simulink library "ConverterLibrary"  (R2026a)
settings: Solver=VariableStepAuto
undefined symbols (not defined in the file or in its folder): DiscIntNeverNeededParam, dspblkCoreblockFVToolHelper, gcbh, gridInverter
libraries: fl_lib x240, nesl_utility x221, ee_lib x208, slpidlib x28, eeGeneralControl x12, simulink x9, eeTransforms x4, simulink_extras x1, eePowerMeasurement x1
(part 6 of 30)

== system ConverterLibrary/Controller/Inverter-Based Resources/Grid-Forming Converter Controller/Measurement ==
  Vgabcc : Inport
  Igabc : Inport  Port=2
  Angle : Inport  Port=3
  Frequency Measurement : Subsystem
  Gain1 : Gain  Gain=1/power
  Gain2 : Gain  Gain=1/power
  Gain3 : Gain  Gain=gridLineVoltage*sqrt(2/3)
  Gain4 : Gain  Gain=gridLineVoltage*sqrt(2/3)
  Gain5 : Gain  Gain=power/(sqrt(3)*gridLineVoltage)*sqrt(2)
  PU2Hz : Gain  Gain=gridInverter.frequency
  Power Measurement (Three-Phase)1 : eePowerMeasurement/Power Measurement (Three-Phase)  LabelModeActiveChoice=Discrete  F=powerFreq  K=[1]  Seq=Positive  Ts=measSampleTime
  abc2dq : Subsystem
  Out Bus Element : Outport  PortName=measure  Element=P
  Out Bus Element1 : Outport  PortName=measure  Element=Q
  Out Bus Element2 : Outport  PortName=measure  Element=Vgd
  Out Bus Element3 : Outport  PortName=measure  Element=Vgq
  Out Bus Element4 : Outport  PortName=measure  Element=Igd
  Out Bus Element5 : Outport  PortName=measure  Element=Igq
  Out Bus Element6 : Outport  PortName=measure  Element=fgrid
  PmeasPU : Outport  Port=2
  QmeasPU : Outport  Port=3
  FmeasHz : Outport  Port=4
  wires:
  Gain3/1 -> Frequency Measurement/1(Vabc)  "Vgd"
  Gain1/1 -> Out Bus Element1/1, QmeasPU/1  "Qmeas"
  Gain2/1 -> PmeasPU/1, Out Bus Element/1  "Pmeas"
  Gain5/1 -> Power Measurement (Three-Phase)1/2  "Igd"
  Gain4/1 -> Power Measurement (Three-Phase)1/1  "Vgd"
  Power Measurement (Three-Phase)1/2 -> Gain1/1  "Qmeas"
  Power Measurement (Three-Phase)1/1 -> Gain2/1  "Pmeas"
  PU2Hz/1 -> FmeasHz/1
  Frequency Measurement/1(freq) -> Out Bus Element6/1, PU2Hz/1
  abc2dq/4(Igq) -> Out Bus Element5/1  "Igq"
  abc2dq/3(Igd) -> Out Bus Element4/1  "Igd"
  abc2dq/1(Vgd) -> Out Bus Element2/1  "Vgd"
  abc2dq/2(Vgq) -> Out Bus Element3/1  "Vgq"
  Igabc/1 -> abc2dq/1(Igabc), Gain5/1  "Iabc"
  Angle/1 -> abc2dq/2(Angle)
  Vgabcc/1 -> Gain4/1, Gain3/1, abc2dq/3(Vgabc)  "Vabc"

== system ConverterLibrary/Controller/Inverter-Based Resources/Grid-Forming Converter Controller/Power Control ==
  note: Active Power Control
  note: Reactive Power Control
  In Bus Element2 : Inport  PortName=measure  Element=P
  In Bus Element3 : Inport  PortName=measure  Element=Q
  In Bus Element1 : Inport  PortName=measure  Element=fgrid
  Pref : Inport  Port=2
  Qref : Inport  Port=3
  ActivePowerControl : Subsystem  Variant=on  VariantControlMode=label  VariantControl=Choice  LabelModeActiveChoice=vsm
  ReactiveControl : Subsystem
  Out Bus Element : Outport  PortName=reactiveControl  Element=Vmd
  Out Bus Element1 : Outport  PortName=reactiveControl  Element=Vmq
  Out Bus Element6 : Outport  Port=2  PortName=activeControl  Element=angle
  Out Bus Element4 : Outport  Port=2  PortName=activeControl  Element=w
  angle : Outport  Port=3
  wires:
  In Bus Element1/1 -> ActivePowerControl/3(fgrid)
  In Bus Element2/1 -> ActivePowerControl/2(Pmeas)
  Qref/1 -> ReactiveControl/1(Qref)  "Q"
  Pref/1 -> ActivePowerControl/1(Pref)  "Q"
  ReactiveControl/2(Vmq) -> Out Bus Element1/1
  ReactiveControl/1(Vmd) -> Out Bus Element/1
  ActivePowerControl/1(Theta) -> Out Bus Element6/1, angle/1
  In Bus Element3/1 -> ReactiveControl/2(Qmeas)
  ActivePowerControl/2(w) -> Out Bus Element4/1

== system ConverterLibrary/Controller/Inverter-Based Resources/Grid-Forming Converter Controller/VoltageCurrentControl ==
  In Bus Element : Inport  PortName=currentLimiting  Element=Vmd
  In Bus Element1 : Inport  PortName=currentLimiting  Element=Vmq
  In Bus Element6 : Inport  PortName=currentLimiting  Element=Idmax
  In Bus Element7 : Inport  PortName=currentLimiting  Element=Iqmax
  Bus Element In6 : Inport  Port=2  PortName=activeControl  Element=w
  Bus Element In1 : Inport  Port=2  PortName=activeControl  Element=angle
  In Bus Element2 : Inport  Port=3  PortName=measure  Element=Vgd
  In Bus Element3 : Inport  Port=3  PortName=measure  Element=Vgq
  In Bus Element4 : Inport  Port=3  PortName=measure  Element=Igd
  In Bus Element5 : Inport  Port=3  PortName=measure  Element=Igq
  Controller : Subsystem
  Modulation Signal : Subsystem
  mabc : Outport
  wires:
  Bus Element In1/1 -> Modulation Signal/3(Angle)
  In Bus Element1/1 -> Controller/3(Vgqref)
  In Bus Element/1 -> Controller/2(Vgdref)
  Bus Element In6/1 -> Controller/1(Angfreq)
  In Bus Element3/1 -> Controller/5(Vsq)
  In Bus Element2/1 -> Controller/4(Vsd)
  In Bus Element7/1 -> Controller/9(Iqmax)
  In Bus Element6/1 -> Controller/8(Idmax)
  In Bus Element5/1 -> Controller/7(Iq)
  In Bus Element4/1 -> Controller/6(Id)
  Controller/1(Vd) -> Modulation Signal/1(Vd)
  Modulation Signal/1(mabc) -> mabc/1
  Controller/2(Vq) -> Modulation Signal/2(Vq)

== system ConverterLibrary/Controller/Non-Isolated DC-DC Converters/Non-Isolated DC-DC Controller/Duty Feedforward ==
  voltageReferencePu : Inport
  inputVoltagePuOut : Inport  Port=2
  Duty Max : Constant  Value=dutyMax
  Duty Min : Constant  Value=dutyMin
  Feedforward Law : Subsystem  Variant=on  VariantControlMode=label  LabelModeActiveChoice=Boost
  Feedforward Limit : Saturate  UpperLimit=dutyMax  LowerLimit=dutyMin
  Input Clamp : Saturate  UpperLimit=inf  LowerLimit=inputVoltagePuMin
  Reference Clamp : Saturate  UpperLimit=inf  LowerLimit=voltageReferencePuMin
  Sum : Sum  Inputs=|+-
  Sum1 : Sum  Inputs=|-+
  trimUpperLimit : Outport
  trimLowerLimit : Outport  Port=2
  dutyFeedforward : Outport  Port=3
  wires:
  Feedforward Limit/1 -> dutyFeedforward/1, Sum1/1, Sum/2
  Feedforward Law/1(dutyFeedforward) -> Feedforward Limit/1
  Input Clamp/1 -> Feedforward Law/2(inputVoltagePuOut)
  Reference Clamp/1 -> Feedforward Law/1(voltageReferencePu)
  inputVoltagePuOut/1 -> Input Clamp/1
  voltageReferencePu/1 -> Reference Clamp/1
  Duty Max/1 -> Sum/1
  Sum/1 -> trimUpperLimit/1
  Sum1/1 -> trimLowerLimit/1
  Duty Min/1 -> Sum1/2

== system ConverterLibrary/Controller/Non-Isolated DC-DC Converters/Non-Isolated DC-DC Controller/Loop Structure ==
  voltageControllerOutput : Inport
  inductorCurrentPu : Inport  Port=2
  trimUpperLimit : Inport  Port=3
  trimLowerLimit : Inport  Port=4
  DoubleLoop : Subsystem  VariantControl=DoubleLoop
  SingleLoop : Subsystem  VariantControl=SingleLoop
  dutyTrim : Outport

== system ConverterLibrary/Controller/Non-Isolated DC-DC Converters/Non-Isolated DC-DC Controller/Output Mode ==
  duty : Inport
  DutyCycle : Subsystem  VariantControl=DutyCycle
  PWMSignal : Subsystem  VariantControl=PWMSignal
  G : Outport

== system ConverterLibrary/Controller/Non-Isolated DC-DC Converters/Non-Isolated DC-DC Controller/Per-Unit Scaling ==
  Vref : Inport
  Vmeas : Inport  Port=2
  Imeas : Inport  Port=3
  Vin : Inport  Port=4
  Imeas ADC Sample : UnitDelay  SampleTime=TsCurrent
  Imeas Inductor Base : Gain  Gain=1/IbaseL
  Vin ADC Sample : UnitDelay  InitialCondition=VbaseIn  SampleTime=TsVoltage
  Vin Output Base : Gain  Gain=1/VbaseOut
  Vmeas ADC Sample : UnitDelay  SampleTime=TsVoltage
  Vmeas Output Base : Gain  Gain=1/VbaseOut
  Vref Output Base : Gain  Gain=1/VbaseOut
  outputVoltagePu : Outport
  voltageReferencePu : Outport  Port=2
  inductorCurrentPu : Outport  Port=3
  inputVoltagePuOut : Outport  Port=4
  wires:
  Vin Output Base/1 -> inputVoltagePuOut/1
  Vin ADC Sample/1 -> Vin Output Base/1
  Vin/1 -> Vin ADC Sample/1
  Imeas Inductor Base/1 -> inductorCurrentPu/1
  Imeas ADC Sample/1 -> Imeas Inductor Base/1
  Imeas/1 -> Imeas ADC Sample/1
  Vmeas Output Base/1 -> outputVoltagePu/1
  Vmeas ADC Sample/1 -> Vmeas Output Base/1
  Vmeas/1 -> Vmeas ADC Sample/1
  Vref Output Base/1 -> voltageReferencePu/1
  Vref/1 -> Vref Output Base/1

== system ConverterLibrary/Controller/Non-Isolated DC-DC Converters/Non-Isolated DC-DC Controller/Voltage Controller ==
  error : Inport
  PIContinuous : Subsystem  VariantControl=PIContinuous
  PIDiscrete : Subsystem  VariantControl=PIDiscrete
  vc : Outport

== system ConverterLibrary/Controller/PWM Generators/CLLC PWM Generator/Primary Gate Signal ==
  fpu : Inport
  Bridge Gate Map : Selector  InputPortWidth=2  IndexOptions=Index vector (dialog)  Indices=[1 2 2 1]  OutputSizes=1
  Dead Time : Constant  Value=Tdead
  Gate Level Offset : Bias  Bias=gateVoltageOff
  Gate Level Swing : Gain  Gain=gateVoltageOn - gateVoltageOff
  Hertz To Period : Math  Operator=reciprocal
  Leg Gate Logic : Subsystem
  Normalized To Hertz : Gain  Gain=Fbase
  Primary Gates To Logic : DataTypeConversion  OutDataTypeStr=boolean
  Pulse Time : Gain  Gain=pulseWidth
  Pulse Time Plus Dead Time : Bias  Bias=Tdead
  Ramp Mode : Subsystem  Variant=on  VariantControlMode=label  LabelModeActiveChoice=VariableStep
  Turn Off Times : Mux  Inputs=2
  Turn On Times : Mux  Inputs=2
  G : Outport
  gates : Outport  Port=2
  wires:
  Gate Level Swing/1 -> Gate Level Offset/1
  fpu/1 -> Normalized To Hertz/1
  Normalized To Hertz/1 -> Hertz To Period/1
  Hertz To Period/1 -> Pulse Time/1, Turn Off Times/2, Ramp Mode/1(Tsw)
  Pulse Time/1 -> Pulse Time Plus Dead Time/1, Turn Off Times/1
  Dead Time/1 -> Turn On Times/1
  Pulse Time Plus Dead Time/1 -> Turn On Times/2
  Turn On Times/1 -> Leg Gate Logic/1(Ton)
  Turn Off Times/1 -> Leg Gate Logic/2(Toff)
  Ramp Mode/1(S) -> Leg Gate Logic/3(S)
  Leg Gate Logic/1(gates) -> Bridge Gate Map/1
  Bridge Gate Map/1 -> Gate Level Swing/1, Primary Gates To Logic/1
  Gate Level Offset/1 -> G/1
  Primary Gates To Logic/1 -> gates/1

== system ConverterLibrary/Controller/PWM Generators/CLLC PWM Generator/Synchronous Rectifier ==
  primaryGates : Inport
  fpu : Inport  Port=2
  Isec : Inport  Port=3
  Conduction Detect : Subsystem
  Rectifier Gate Level Offset : Bias  Bias=srGateVoltageOff
  Rectifier Gate Level Swing : Gain  Gain=srGateVoltageOn - srGateVoltageOff
  Rectifier Gates To Double : DataTypeConversion  OutDataTypeStr=double
  Region Select : Subsystem
  Turn On Delay : Subsystem
  Gs : Outport
  wires:
  Rectifier Gate Level Swing/1 -> Rectifier Gate Level Offset/1
  primaryGates/1 -> Region Select/1(primaryGates)
  fpu/1 -> Region Select/2(fpu)
  Isec/1 -> Conduction Detect/1(Isec)
  Conduction Detect/1(permit) -> Region Select/3(permit)
  Region Select/1(Gs) -> Turn On Delay/1(condition)
  Turn On Delay/1(Gs) -> Rectifier Gates To Double/1
  Rectifier Gates To Double/1 -> Rectifier Gate Level Swing/1
  Rectifier Gate Level Offset/1 -> Gs/1

== system ConverterLibrary/Controller/PWM Generators/Complementary PWM Generator/Ramp Mode ==
  rate : Inport
  FixedStep : Subsystem  VariantControl=FixedStep
  VariableStep : Subsystem  VariantControl=VariableStep
  S : Outport

== system ConverterLibrary/Controller/PWM Generators/DAB PWM Generator/Primary Leg Gate Logic ==
  Ton : Inport
  Toff : Inport  Port=2
  S : Inport  Port=3
  After Turn Off : RelationalOperator
  After Turn On : RelationalOperator
  Pulse Window : Logic  Operator=XOR
  To Double : DataTypeConversion  OutDataTypeStr=double
  gates : Outport
  wires:
  Ton/1 -> After Turn On/2
  Toff/1 -> After Turn Off/2
  S/1 -> After Turn Off/1, After Turn On/1
  After Turn On/1 -> Pulse Window/1
  After Turn Off/1 -> Pulse Window/2
  Pulse Window/1 -> To Double/1
  To Double/1 -> gates/1

== system ConverterLibrary/Controller/PWM Generators/DAB PWM Generator/Ramp Mode ==
  Tsw : Inport
  FixedStep : Subsystem  VariantControl=FixedStep
  VariableStep : Subsystem  VariantControl=VariableStep
  S : Outport

== system ConverterLibrary/Controller/PWM Generators/DAB PWM Generator/Secondary Leg Gate Logic ==
  Ton : Inport
  Toff : Inport  Port=2
  S : Inport  Port=3
  After Turn Off : RelationalOperator
  After Turn On : RelationalOperator
  Pulse Window : Logic  Operator=XOR
  To Double : DataTypeConversion  OutDataTypeStr=double
  gates : Outport
  wires:
  Ton/1 -> After Turn On/2
  Toff/1 -> After Turn Off/2
  S/1 -> After Turn Off/1, After Turn On/1
  After Turn On/1 -> Pulse Window/1
  After Turn Off/1 -> Pulse Window/2
  Pulse Window/1 -> To Double/1
  To Double/1 -> gates/1

== system ConverterLibrary/Controller/PWM Generators/Full Bridge PWM Generator/Leg Gate Logic ==
  Ton : Inport
  Toff : Inport  Port=2
  S : Inport  Port=3
  After Turn Off : RelationalOperator
  After Turn On : RelationalOperator
  Pulse Window : Logic  Operator=XOR
  To Double : DataTypeConversion  OutDataTypeStr=double
  gates : Outport
  wires:
  Ton/1 -> After Turn On/2
  Toff/1 -> After Turn Off/2
  S/1 -> After Turn Off/1, After Turn On/1
  After Turn On/1 -> Pulse Window/1
  After Turn Off/1 -> Pulse Window/2
  Pulse Window/1 -> To Double/1
  To Double/1 -> gates/1

== system ConverterLibrary/Controller/PWM Generators/Full Bridge PWM Generator/Ramp Mode ==
  Tsw : Inport
  FixedStep : Subsystem  VariantControl=FixedStep
  VariableStep : Subsystem  VariantControl=VariableStep
  S : Outport

== system ConverterLibrary/Controller/PWM Generators/Half Bridge PWM Generator/Leg Gate Logic ==
  Ton : Inport
  Toff : Inport  Port=2
  S : Inport  Port=3
  After Turn Off : RelationalOperator
  After Turn On : RelationalOperator
  Pulse Window : Logic  Operator=XOR
  To Double : DataTypeConversion  OutDataTypeStr=double
  gates : Outport
  wires:
  Ton/1 -> After Turn On/2
  Toff/1 -> After Turn Off/2
  S/1 -> After Turn Off/1, After Turn On/1
  After Turn On/1 -> Pulse Window/1
  After Turn Off/1 -> Pulse Window/2
  Pulse Window/1 -> To Double/1
  To Double/1 -> gates/1

== system ConverterLibrary/Controller/PWM Generators/Half Bridge PWM Generator/Ramp Mode ==
  Tsw : Inport
  FixedStep : Subsystem  VariantControl=FixedStep
  VariableStep : Subsystem  VariantControl=VariableStep
  S : Outport

== system ConverterLibrary/Controller/PWM Generators/LLC PWM Generator/Leg Gate Logic ==
  Ton : Inport
  Toff : Inport  Port=2
  S : Inport  Port=3
  After Turn Off : RelationalOperator
  After Turn On : RelationalOperator
  Pulse Window : Logic  Operator=XOR
  To Double : DataTypeConversion  OutDataTypeStr=double
  gates : Outport
  wires:
  Ton/1 -> After Turn On/2
  Toff/1 -> After Turn Off/2
  S/1 -> After Turn Off/1, After Turn On/1
  After Turn On/1 -> Pulse Window/1
  After Turn Off/1 -> Pulse Window/2
  Pulse Window/1 -> To Double/1
  To Double/1 -> gates/1

== system ConverterLibrary/Controller/PWM Generators/LLC PWM Generator/Ramp Mode ==
  Tsw : Inport
  FixedStep : Subsystem  VariantControl=FixedStep
  VariableStep : Subsystem  VariantControl=VariableStep
  S : Outport

== system ConverterLibrary/Controller/Power Factor Correction Converters/Boost PFC Controller/Current Controller ==
  error : Inport
  up : Inport  Port=2
  lo : Inport  Port=3
  PIContinuous : Subsystem  VariantControl=PIContinuous
  PIDiscrete : Subsystem  VariantControl=PIDiscrete
  vc : Outport

== system ConverterLibrary/Controller/Power Factor Correction Converters/Boost PFC Controller/Duty Feedforward ==
  busVoltagePuDC : Inport
  absLineVoltagePuDC : Inport  Port=2
  Bus Clamp : Saturate  UpperLimit=inf  LowerLimit=VacPeakPuDC
  Duty Max : Constant  Value=dutyMax
  Duty Min : Constant  Value=dutyMin
  Feedforward One : Constant
  Feedforward Ratio : Product  Inputs=*/
  One Minus Ratio : Sum  Inputs=|+-
  Trim Lower Limit : Sum  Inputs=|+-
  Trim Upper Limit : Sum  Inputs=|+-
  trimUpperLimit : Outport
  trimLowerLimit : Outport  Port=2
  dutyFeedforward : Outport  Port=3
  wires:
  Trim Lower Limit/1 -> trimLowerLimit/1
  Trim Upper Limit/1 -> trimUpperLimit/1
  Duty Min/1 -> Trim Lower Limit/1
  Duty Max/1 -> Trim Upper Limit/1
  One Minus Ratio/1 -> Trim Lower Limit/2, Trim Upper Limit/2, dutyFeedforward/1
  Feedforward Ratio/1 -> One Minus Ratio/2
  Feedforward One/1 -> One Minus Ratio/1
  Bus Clamp/1 -> Feedforward Ratio/2
  absLineVoltagePuDC/1 -> Feedforward Ratio/1
  busVoltagePuDC/1 -> Bus Clamp/1

== system ConverterLibrary/Controller/Power Factor Correction Converters/Boost PFC Controller/Output Mode ==
  duty : Inport
  DutyCycle : Subsystem  VariantControl=DutyCycle
  PWMSignal : Subsystem  VariantControl=PWMSignal
  G : Outport

== system ConverterLibrary/Controller/Power Factor Correction Converters/Boost PFC Controller/Per-Unit Scaling ==
  Vac : Inport
  Vref : Inport  Port=2
  Vmeas : Inport  Port=3
  IL : Inport  Port=4
  Abs Line Current : Abs  SaturateOnIntegerOverflow=off
  Abs Vac : Abs  SaturateOnIntegerOverflow=off
  Abs Vac AC Base : Gain  Gain=1/VbaseAC
  Abs Vac DC Base : Gain  Gain=1/VbaseDC
  IL AC Base : Gain  Gain=1/IbaseAC
  IL ADC Sample : UnitDelay  SampleTime=TsCurrent
  Vac ADC Sample : UnitDelay  SampleTime=TsCurrent
  Vmeas ADC Sample : UnitDelay  SampleTime=TsVoltage
  Vmeas DC Base : Gain  Gain=1/VbaseDC
  Vref DC Base : Gain  Gain=1/VbaseDC
  absLineVoltagePuAC : Outport
  voltageReferencePuDC : Outport  Port=2
  busVoltagePuDC : Outport  Port=3
  absLineCurrentPuAC : Outport  Port=4
  absLineVoltagePuDC : Outport  Port=5
  wires:
  Abs Line Current/1 -> absLineCurrentPuAC/1
  IL AC Base/1 -> Abs Line Current/1
  IL ADC Sample/1 -> IL AC Base/1
  IL/1 -> IL ADC Sample/1
  Vmeas DC Base/1 -> busVoltagePuDC/1
  Vmeas ADC Sample/1 -> Vmeas DC Base/1
  Vmeas/1 -> Vmeas ADC Sample/1
  Vref DC Base/1 -> voltageReferencePuDC/1
  Vref/1 -> Vref DC Base/1
  Abs Vac DC Base/1 -> absLineVoltagePuDC/1
  Abs Vac AC Base/1 -> absLineVoltagePuAC/1
  Abs Vac/1 -> Abs Vac AC Base/1, Abs Vac DC Base/1
  Vac ADC Sample/1 -> Abs Vac/1
  Vac/1 -> Vac ADC Sample/1

== system ConverterLibrary/Controller/Power Factor Correction Converters/Boost PFC Controller/Voltage Controller ==
  error : Inport
  PIContinuous : Subsystem  VariantControl=PIContinuous
  PIDiscrete : Subsystem  VariantControl=PIDiscrete
  vc : Outport

== system ConverterLibrary/Controller/Power Factor Correction Converters/Interleaved Boost PFC Controller/Current Balance ==
  leg1CurrentPuAC : Inport
  leg2CurrentPuAC : Inport  Port=2
  Balance Controller : Subsystem  Variant=on  VariantControlMode=label  LabelModeActiveChoice=PIContinuous
  Half Difference : Gain  Gain=0.5
  Leg Current Difference : Sum  Inputs=|+-
  dutyTrim : Outport
  wires:
  Balance Controller/1(vc) -> dutyTrim/1
  Half Difference/1 -> Balance Controller/1(error)
  Leg Current Difference/1 -> Half Difference/1
  leg2CurrentPuAC/1 -> Leg Current Difference/2
  leg1CurrentPuAC/1 -> Leg Current Difference/1

== system ConverterLibrary/Controller/Power Factor Correction Converters/Interleaved Boost PFC Controller/Current Controller ==
  error : Inport
  up : Inport  Port=2
  lo : Inport  Port=3
  PIContinuous : Subsystem  VariantControl=PIContinuous
  PIDiscrete : Subsystem  VariantControl=PIDiscrete
  vc : Outport

== system ConverterLibrary/Controller/Power Factor Correction Converters/Interleaved Boost PFC Controller/Duty Feedforward ==
  busVoltagePuDC : Inport
  absLineVoltagePuDC : Inport  Port=2
  Bus Clamp : Saturate  UpperLimit=inf  LowerLimit=VacPeakPuDC
  Duty Max : Constant  Value=dutyMax
  Duty Min : Constant  Value=dutyMin
  Feedforward One : Constant
  Feedforward Ratio : Product  Inputs=*/
  One Minus Ratio : Sum  Inputs=|+-
  Trim Lower Limit : Sum  Inputs=|+-
  Trim Upper Limit : Sum  Inputs=|+-
  trimUpperLimit : Outport
  trimLowerLimit : Outport  Port=2
  dutyFeedforward : Outport  Port=3
  wires:
  Trim Lower Limit/1 -> trimLowerLimit/1
  Trim Upper Limit/1 -> trimUpperLimit/1
  Duty Min/1 -> Trim Lower Limit/1
  Duty Max/1 -> Trim Upper Limit/1
  One Minus Ratio/1 -> dutyFeedforward/1, Trim Upper Limit/2, Trim Lower Limit/2
  Feedforward Ratio/1 -> One Minus Ratio/2
  Feedforward One/1 -> One Minus Ratio/1
  Bus Clamp/1 -> Feedforward Ratio/2
  absLineVoltagePuDC/1 -> Feedforward Ratio/1
  busVoltagePuDC/1 -> Bus Clamp/1

== system ConverterLibrary/Controller/Power Factor Correction Converters/Interleaved Boost PFC Controller/Duty Split ==
  dutyCommon : Inport
  dutyTrim : Inport  Port=2
  Leg 1 Duty : Sum  Inputs=|+-
  Leg 1 Duty Limit : Saturate  UpperLimit=dutyMax  LowerLimit=dutyMin
  Leg 2 Duty : Sum  Inputs=|++
  Leg 2 Duty Limit : Saturate  UpperLimit=dutyMax  LowerLimit=dutyMin
  Leg Duties : Mux  Inputs=2
  duty : Outport
  wires:
  Leg Duties/1 -> duty/1
  Leg 2 Duty Limit/1 -> Leg Duties/2
  Leg 1 Duty Limit/1 -> Leg Duties/1
  Leg 2 Duty/1 -> Leg 2 Duty Limit/1
  Leg 1 Duty/1 -> Leg 1 Duty Limit/1
  dutyTrim/1 -> Leg 2 Duty/2, Leg 1 Duty/2
  dutyCommon/1 -> Leg 2 Duty/1, Leg 1 Duty/1

== system ConverterLibrary/Controller/Power Factor Correction Converters/Interleaved Boost PFC Controller/Output Mode ==
  duty : Inport
  DutyCycle : Subsystem  VariantControl=DutyCycle
  PWMSignal : Subsystem  VariantControl=PWMSignal
  G : Outport

== system ConverterLibrary/Controller/Power Factor Correction Converters/Interleaved Boost PFC Controller/Per-Unit Scaling ==
  Vac : Inport
  Vref : Inport  Port=2
  Vmeas : Inport  Port=3
  IL1 : Inport  Port=4
  IL2 : Inport  Port=5
  Abs Line Current : Abs  SaturateOnIntegerOverflow=off
  Abs Vac : Abs  SaturateOnIntegerOverflow=off
  Abs Vac AC Base : Gain  Gain=1/VbaseAC
  Abs Vac DC Base : Gain  Gain=1/VbaseDC
  IL1 AC Base : Gain  Gain=1/IbaseAC
  IL1 ADC Sample : UnitDelay  SampleTime=TsCurrent
  IL2 AC Base : Gain  Gain=1/IbaseAC
  IL2 ADC Sample : UnitDelay  SampleTime=TsCurrent
  Total Line Current : Sum  Inputs=|++
  Vac ADC Sample : UnitDelay  SampleTime=TsCurrent
  Vmeas ADC Sample : UnitDelay  SampleTime=TsVoltage
  Vmeas DC Base : Gain  Gain=1/VbaseDC
  Vref DC Base : Gain  Gain=1/VbaseDC
  absLineCurrentPuAC : Outport
  absLineVoltagePuAC : Outport  Port=2
  voltageReferencePuDC : Outport  Port=3
  busVoltagePuDC : Outport  Port=4
  absLineVoltagePuDC : Outport  Port=5
  leg1CurrentPuAC : Outport  Port=6
  leg2CurrentPuAC : Outport  Port=7
  wires:
  Abs Line Current/1 -> absLineCurrentPuAC/1
  Total Line Current/1 -> Abs Line Current/1
  IL2 AC Base/1 -> leg2CurrentPuAC/1, Total Line Current/2
  IL1 AC Base/1 -> leg1CurrentPuAC/1, Total Line Current/1
  IL2 ADC Sample/1 -> IL2 AC Base/1
  IL2/1 -> IL2 ADC Sample/1
  IL1 ADC Sample/1 -> IL1 AC Base/1
  IL1/1 -> IL1 ADC Sample/1
  Vmeas DC Base/1 -> busVoltagePuDC/1
  Vmeas ADC Sample/1 -> Vmeas DC Base/1
  Vmeas/1 -> Vmeas ADC Sample/1
  Vref DC Base/1 -> voltageReferencePuDC/1
  Vref/1 -> Vref DC Base/1
  Abs Vac DC Base/1 -> absLineVoltagePuDC/1
  Abs Vac AC Base/1 -> absLineVoltagePuAC/1
  Abs Vac/1 -> Abs Vac AC Base/1, Abs Vac DC Base/1
  Vac ADC Sample/1 -> Abs Vac/1
  Vac/1 -> Vac ADC Sample/1

== system ConverterLibrary/Controller/Power Factor Correction Converters/Interleaved Boost PFC Controller/Voltage Controller ==
  error : Inport
  PIContinuous : Subsystem  VariantControl=PIContinuous
  PIDiscrete : Subsystem  VariantControl=PIDiscrete
  vc : Outport

== system ConverterLibrary/Controller/Power Factor Correction Converters/Totem-Pole Boost PFC Controller/Current Controller ==
  note: 1) Add Subsystem or Model blocks as valid variant choices.
      | 2) You cannot connect blocks at this level. At simulation, connectivity is automatically
      | determined, based on the active variant and port name matching.
  error : Inport
  up : Inport  Port=2
  lo : Inport  Port=3
  PIContinuous : Subsystem  VariantControl=PIContinuous
  PIDiscrete : Subsystem  VariantControl=PIDiscrete
  vc : Outport

== system ConverterLibrary/Controller/Power Factor Correction Converters/Totem-Pole Boost PFC Controller/Duty Feedforward ==
  busVoltagePuDC : Inport
  absLineVoltagePuDC : Inport  Port=2
  Bus Clamp : Saturate  UpperLimit=inf  LowerLimit=VacPeakPuDC
  Duty Max : Constant  Value=dutyMax
  Duty Min : Constant  Value=dutyMin
  Feedforward One : Constant
  Feedforward Ratio : Product  Inputs=*/
  One Minus Ratio : Sum  Inputs=+-
  Trim Lower Limit : Sum  Inputs=+-
  Trim Upper Limit : Sum  Inputs=+-
  trimUpperLimit : Outport
  trimLowerLimit : Outport  Port=2
  dutyFeedforward : Outport  Port=3
  wires:
  Trim Lower Limit/1 -> trimLowerLimit/1
  Trim Upper Limit/1 -> trimUpperLimit/1
  Duty Min/1 -> Trim Lower Limit/1
  Duty Max/1 -> Trim Upper Limit/1
  One Minus Ratio/1 -> dutyFeedforward/1, Trim Lower Limit/2, Trim Upper Limit/2
  Feedforward Ratio/1 -> One Minus Ratio/2
  Feedforward One/1 -> One Minus Ratio/1
  Bus Clamp/1 -> Feedforward Ratio/2
  absLineVoltagePuDC/1 -> Feedforward Ratio/1
  busVoltagePuDC/1 -> Bus Clamp/1

== system ConverterLibrary/Controller/Power Factor Correction Converters/Totem-Pole Boost PFC Controller/Gate Logic ==
  u : Inport
  Vac : Inport  Port=2
  Demux : Demux  Outputs=2
  Line Polarity : Switch  SaturateOnIntegerOverflow=off  InputSameDT=off
  Negative Half Gates : Selector  InputPortWidth=4  IndexOptions=Index vector (dialog)  Indices=[2 1 3 4]  OutputSizes=1
  Positive Half Gates : Mux
  Selector : Selector  InputPortWidth=2  IndexOptions=Index vector (dialog)  Indices=[2 1]  OutputSizes=1
  Slow Leg Complementary PWM : Subsystem
  Slow Leg Gate Order : Selector  InputPortWidth=2  IndexOptions=Index vector (dialog)  Indices=[2 1]  OutputSizes=1
  Slow Leg Gates : Demux  Outputs=2
  G : Outport
  wires:
  Slow Leg Gates/2 -> Positive Half Gates/4
  Slow Leg Gates/1 -> Positive Half Gates/3
  Slow Leg Gate Order/1 -> Slow Leg Gates/1
  Slow Leg Complementary PWM/1(G) -> Slow Leg Gate Order/1
  Selector/1 -> Demux/1
  Demux/2 -> Positive Half Gates/2
  Demux/1 -> Positive Half Gates/1
  u/1 -> Selector/1
  Positive Half Gates/1 -> Negative Half Gates/1, Line Polarity/1
  Vac/1 -> Line Polarity/2, Slow Leg Complementary PWM/1(PWM)
  Negative Half Gates/1 -> Line Polarity/3
  Line Polarity/1 -> G/1

== system ConverterLibrary/Controller/Power Factor Correction Converters/Totem-Pole Boost PFC Controller/Output Mode ==
  duty : Inport
  DutyCycle : Subsystem  VariantControl=DutyCycle
  PWMSignal : Subsystem  VariantControl=PWMSignal
  G : Outport

== system ConverterLibrary/Controller/Power Factor Correction Converters/Totem-Pole Boost PFC Controller/Per-Unit Scaling ==
  Vac : Inport
  Vref : Inport  Port=2
  Vmeas : Inport  Port=3
  Imeas : Inport  Port=4
  Abs Imeas : Abs
  Abs Vac : Abs
  Abs Vac AC Base : Gain  Gain=1/VbaseAC
  Abs Vac DC Base : Gain  Gain=1/VbaseDC
  Imeas AC Base : Gain  Gain=1/IbaseAC
  Imeas ADC Sample : UnitDelay  SampleTime=TsCurrent
  Vac AC Base : Gain  Gain=1/VbaseAC
  Vac ADC Sample : UnitDelay  SampleTime=TsCurrent
  Vmeas ADC Sample : UnitDelay  SampleTime=TsVoltage
  Vmeas DC Base : Gain  Gain=1/VbaseDC
  Vref DC Base : Gain  Gain=1/VbaseDC
  absLineVoltagePuAC : Outport
  voltageReferencePuDC : Outport  Port=2
  busVoltagePuDC : Outport  Port=3
  absLineCurrentPuAC : Outport  Port=4
  absLineVoltagePuDC : Outport  Port=5
  lineVoltagePuAC : Outport  Port=6
  wires:
  Imeas AC Base/1 -> absLineCurrentPuAC/1
  Abs Imeas/1 -> Imeas AC Base/1
  Imeas ADC Sample/1 -> Abs Imeas/1
  Imeas/1 -> Imeas ADC Sample/1
  Vmeas DC Base/1 -> busVoltagePuDC/1
  Vmeas ADC Sample/1 -> Vmeas DC Base/1
  Vmeas/1 -> Vmeas ADC Sample/1
  Vref DC Base/1 -> voltageReferencePuDC/1
  Vref/1 -> Vref DC Base/1
  Abs Vac DC Base/1 -> absLineVoltagePuDC/1
  Vac AC Base/1 -> lineVoltagePuAC/1
  Abs Vac AC Base/1 -> absLineVoltagePuAC/1
  Abs Vac/1 -> Abs Vac DC Base/1, Abs Vac AC Base/1
  Vac ADC Sample/1 -> Abs Vac/1, Vac AC Base/1
  Vac/1 -> Vac ADC Sample/1

== system ConverterLibrary/Controller/Power Factor Correction Converters/Totem-Pole Boost PFC Controller/Voltage Controller ==
  note: 1) Add Subsystem or Model blocks as valid variant choices.
      | 2) You cannot connect blocks at this level. At simulation, connectivity is automatically
      | determined, based on the active variant and port name matching.
  error : Inport
  PIContinuous : Subsystem  VariantControl=PIContinuous
  PIDiscrete : Subsystem  VariantControl=PIDiscrete
  vc : Outport

== system ConverterLibrary/Controller/Soft-Switching Converters/CLLC Controller/2P2Z Compensator ==
  error : Inport
  CompensatorSDomain : Subsystem  VariantControl=SCompensator
  CompensatorZDomain : Subsystem  VariantControl=ZCompensator
  PIContinuous : Subsystem  VariantControl=PIContinuous
  PIDiscrete : Subsystem  VariantControl=PIDiscrete
  vc : Outport

== system ConverterLibrary/Controller/Soft-Switching Converters/CLLC Controller/Gate Signal ==
  f : Inport
  mode : Inport  Port=2
  Isecondary : Inport  Port=3
  Iprimary : Inport  Port=4
  CLLC PWM Generator : Subsystem
  Rate Transition : RateTransition
  Switch : Switch  Criteria=u2 > Threshold  SaturateOnIntegerOverflow=off  InputSameDT=off
  Switch1 : Switch  Criteria=u2 > Threshold  SaturateOnIntegerOverflow=off  InputSameDT=off
  Switch2 : Switch  Criteria=u2 > Threshold  SaturateOnIntegerOverflow=off  InputSameDT=off
  G1 : Outport
  G2 : Outport  Port=2
  wires:
  CLLC PWM Generator/2(G2) -> Switch2/1, Switch1/3  "cllcRectifierGates"
  CLLC PWM Generator/1(G1) -> Switch1/1, Switch2/3  "cllcPrimaryGates"
  Rate Transition/1 -> CLLC PWM Generator/2(Isec)
  f/1 -> CLLC PWM Generator/1(fpu)
  Iprimary/1 -> Switch/3
  Isecondary/1 -> Switch/1
  mode/1 -> Switch/2, Switch1/2, Switch2/2
  Switch2/1 -> G2/1
  Switch1/1 -> G1/1
  Switch/1 -> Rate Transition/1

== system ConverterLibrary/Controller/Soft-Switching Converters/CLLC Controller/VCO ==
  vc : Inport
  ConstantRate : Subsystem  VariantControl=Constant
  TwoRate : Subsystem  VariantControl=TwoRate
  f : Outport

== system ConverterLibrary/Controller/Soft-Switching Converters/CLLC Controller/Voltage Controller ==
  Ref : Inport
  Vmeas : Inport  Port=2
  Imeas : Inport  Port=3
  CCCV : Inport  Port=4
  Gain1 : Gain  Gain=VdcValue/ratedPower
  If : If  IfExpression=u1 > 0.5  SampleTime=gatingSampleTime
  If Action Subsystem : Subsystem  TreatAsAtomicUnit=on
  If Action Subsystem1 : Subsystem  TreatAsAtomicUnit=on
  Merge : Merge
  Rate Transition : RateTransition
  Rate Transition1 : RateTransition
  Sum : Sum  Inputs=|-+
  Ierr : Outport
  wires:
  Rate Transition1/1 -> If Action Subsystem1/2(Vmeas)
  Rate Transition/1 -> If/1
  Gain1/1 -> Sum/2
  Imeas/1 -> Gain1/1
  Sum/1 -> Ierr/1
  Merge/1 -> Sum/1
  Vmeas/1 -> Rate Transition1/1
  If Action Subsystem1/1(IrefPU) -> Merge/2
  If Action Subsystem/1(Out1) -> Merge/1
  If/2 -> If Action Subsystem1/Action
  If/1 -> If Action Subsystem/Action
  CCCV/1 -> Rate Transition/1
  Ref/1 -> If Action Subsystem/1(Ref), If Action Subsystem1/1(Vref)

== system ConverterLibrary/Controller/Soft-Switching Converters/DAB Controller (SPS)/CC-CV Control ==
  Ref : Inport
  Vmeas : Inport  Port=2
  Imeas : Inport  Port=3
  CCCV : Inport  Port=4
  CC Mode : Subsystem  TreatAsAtomicUnit=on
  CV Mode : Subsystem  TreatAsAtomicUnit=on
  If : If  IfExpression=u1 > 0.5  SampleTime=gatingSampleTimeForControllerType(cntrlSelect, Ts)
  Merge : Merge
  Rate Transition{,1..4} (5 alike) : RateTransition
  phaseShift : Outport
  wires:
  Rate Transition4/1 -> CV Mode/1(Vref)
  CC Mode/1(phaseShift) -> Merge/1
  CV Mode/1(phaseShift) -> Merge/2
  Merge/1 -> phaseShift/1
  Rate Transition3/1 -> CC Mode/2(Imeas)
  CCCV/1 -> Rate Transition/1
  If/1 -> CC Mode/Action
  If/2 -> CV Mode/Action
  Ref/1 -> Rate Transition1/1
  Vmeas/1 -> Rate Transition2/1
  Imeas/1 -> Rate Transition3/1
  Rate Transition/1 -> If/1
  Rate Transition1/1 -> Rate Transition4/1, CC Mode/1(Ref)
  Rate Transition2/1 -> CV Mode/2(Vmeas)

== system ConverterLibrary/Controller/Soft-Switching Converters/DAB Controller (SPS)/Output Mode ==
  phaseShift : Inport
  DutyCycle : Subsystem  VariantControl=DutyCycle
  PWMSignal : Subsystem  VariantControl=PWMSignal
  G1 : Outport
  G2 : Outport  Port=2

== system ConverterLibrary/Controller/Soft-Switching Converters/LLC Voltage Controller/2P2Z Compensator ==
  error : Inport
  CompensatorSDomain : Subsystem  VariantControl=SCompensator
  CompensatorZDomain : Subsystem  VariantControl=ZCompensator
  PIContinuous : Subsystem  VariantControl=PIContinuous
  PIDiscrete : Subsystem  VariantControl=PIDiscrete
  vc : Outport

== system ConverterLibrary/Controller/Soft-Switching Converters/LLC Voltage Controller/LLC PWM Generator ==
  fpu : Inport
  Bridge Gate Map : Selector  InputPortWidth=2  IndexOptions=Index vector (dialog)  Indices=[1 2 2 1]  OutputSizes=1
  Dead Time : Constant  Value=Tdead
  Frequency Limit : Saturate  UpperLimit=(Fmax)  LowerLimit=(Fmin)
  Gate Level Offset : Bias  Bias=(0)
  Gate Level Swing : Gain  Gain=(10) - (0)
  Hertz To Period : Math  Operator=reciprocal
  Leg Gate Logic : Subsystem
  Normalized To Hertz : Gain  Gain=(resFreq)
  Pulse Time : Gain  Gain=(0.5)
  Pulse Time Plus Dead Time : Bias  Bias=Tdead
  Ramp Mode : Subsystem  Variant=on  VariantControlMode=label  LabelModeActiveChoice=VariableStep
  Turn Off Times : Mux  Inputs=2
  Turn On Times : Mux  Inputs=2
  G : Outport
  wires:
  Gate Level Swing/1 -> Gate Level Offset/1
  fpu/1 -> Frequency Limit/1
  Frequency Limit/1 -> Normalized To Hertz/1
  Normalized To Hertz/1 -> Hertz To Period/1
  Hertz To Period/1 -> Pulse Time/1, Turn Off Times/2, Ramp Mode/1(Tsw)
  Pulse Time/1 -> Pulse Time Plus Dead Time/1, Turn Off Times/1
  Dead Time/1 -> Turn On Times/1
  Pulse Time Plus Dead Time/1 -> Turn On Times/2
  Turn On Times/1 -> Leg Gate Logic/1(Ton)
  Turn Off Times/1 -> Leg Gate Logic/2(Toff)
  Ramp Mode/1(S) -> Leg Gate Logic/3(S)
  Leg Gate Logic/1(gates) -> Bridge Gate Map/1
  Bridge Gate Map/1 -> Gate Level Swing/1
  Gate Level Offset/1 -> G/1

== system ConverterLibrary/Controller/Soft-Switching Converters/LLC Voltage Controller/VCO ==
  vc : Inport
  ConstantRate : Subsystem  VariantControl=Constant
  TwoRate : Subsystem  VariantControl=TwoRate
  f : Outport

== system ConverterLibrary/Power Converter Plant/Non-Isolated DC-DC Converters/Non-Isolated DC-DC Converter/NonIsolatedDCDCVariant ==
  G : Inport
  Boost : Subsystem  VariantControl=Boost
  Buck : Subsystem  VariantControl=Buck
  BuckBoost : Subsystem  VariantControl=BuckBoost
  SynchronousBoost : Subsystem  VariantControl=SynchronousBoost
  SynchronousBuck : Subsystem  VariantControl=SynchronousBuck
  SynchronousBuckBoost : Subsystem  VariantControl=SynchronousBuckBoost
  Vin+ : PMIOPort  Side=Left
  Vin- : PMIOPort  Port=2  Side=Left
  Vout+ : PMIOPort  Port=3  Side=Right
  Vout- : PMIOPort  Port=4  Side=Right
  meas : Outport

== system ConverterLibrary/Power Converter Plant/Power Factor Correction Converters/Boost PFC Converter/BoostPFCVariant ==
  G : Inport
  DetailedModel : Subsystem  VariantControl=DetailedModel
  SimplifiedModel : Subsystem  VariantControl=SimplifiedModel
  P : PMIOPort  Side=Left
  N : PMIOPort  Port=2  Side=Left
  + : PMIOPort  Port=3  Side=Right
  - : PMIOPort  Port=4  Side=Right
  meas : Outport

== system ConverterLibrary/Power Converter Plant/Power Factor Correction Converters/Interleaved Boost PFC Converter/InterleavedBoostPFCVariant ==
  G : Inport
  DetailedModel : Subsystem  VariantControl=DetailedModel
  SimplifiedModel : Subsystem  VariantControl=SimplifiedModel
  P : PMIOPort  Side=Left
  N : PMIOPort  Port=2  Side=Left
  + : PMIOPort  Port=3  Side=Right
  - : PMIOPort  Port=4  Side=Right
  meas : Outport

== system ConverterLibrary/Power Converter Plant/Power Factor Correction Converters/Totem-Pole Boost PFC Converter/TotemPoleBoostPFCVariant ==
  G : Inport
  DetailedModel : Subsystem  VariantControl=DetailedModel
  SimplifiedModel : Subsystem  VariantControl=SimplifiedModel
  P : PMIOPort  Side=Left
  N : PMIOPort  Port=2  Side=Left
  + : PMIOPort  Port=3  Side=Right
  - : PMIOPort  Port=4  Side=Right
  meas : Outport

== system ConverterLibrary/Power Converter Plant/Soft-Switching Converters/CLLC Converter/CLLCConverterVariant ==
  Gpri : Inport
  Gsec : Inport  Port=2
  DetailedModel : Subsystem  VariantControl=DetailedModel
  SimplifiedModel : Subsystem  VariantControl=SimplifiedModel
  P1 : PMIOPort  Side=Left
  P2 : PMIOPort  Port=2  Side=Right
  N1 : PMIOPort  Port=3  Side=Left
  N2 : PMIOPort  Port=4  Side=Right
  Meas : Outport

== system ConverterLibrary/Power Converter Plant/Soft-Switching Converters/DAB Converter/DABConverterVariant ==
  Gp : Inport
  Gs : Inport  Port=2
  DetailedModel : Subsystem  VariantControl=DetailedModel
      settings: PortSchema="{\"entries\":[{\"content\":{\"sides\":[{\"content\":{\"connectorIds\":[\"In1\",\"LConn1\",\"LConn2\"]},\"type\":\"ConnectorPlacement.EquallySpacedRectSide\",\"uuid\":\"6f245ee7-ecea-433e-8ace-55b7238b8bbd\"},{\"content\":{\"connectorIds\":[\"In2\",\"Out1\",\"RConn1\",\"RConn2\"],\"side\":\"RIGHT\"},\"type\":\"ConnectorPlacement.EquallySpacedRectSide\",\"uuid\":\"af7f8c88-8cd1-4285-8228-b98ea57f06ae\"},{\"content\":{\"side\":\"TOP\"},\"type\":\"ConnectorPlacement.EquallySpacedRectSide\",\"uuid\":\"820d378e-11b2-4797-9989-1ab18f65f7f5\"}]},\"type\":\"ConnectorPlacement.EquallySpacedConnector\",\"uuid\":\"ae0f71da-cdc3-4120-89e7-21ff59b441bf\"}],\"packageUris\":[\"http://schema.mathworks.com/mf0/Connector/R2020b\"],\"version\":\"1.0\"}"
  SimplifiedModel : Subsystem  VariantControl=SimplifiedModel
      settings: PortSchema="{\"entries\":[{\"content\":{\"sides\":[{\"content\":{\"connectorIds\":[\"In1\",\"LConn1\",\"LConn2\"]},\"type\":\"ConnectorPlacement.EquallySpacedRectSide\",\"uuid\":\"6f245ee7-ecea-433e-8ace-55b7238b8bbd\"},{\"content\":{\"connectorIds\":[\"In2\",\"Out1\",\"RConn1\",\"RConn2\"],\"side\":\"RIGHT\"},\"type\":\"ConnectorPlacement.EquallySpacedRectSide\",\"uuid\":\"af7f8c88-8cd1-4285-8228-b98ea57f06ae\"},{\"content\":{\"side\":\"TOP\"},\"type\":\"ConnectorPlacement.EquallySpacedRectSide\",\"uuid\":\"820d378e-11b2-4797-9989-1ab18f65f7f5\"}]},\"type\":\"ConnectorPlacement.EquallySpacedConnector\",\"uuid\":\"ae0f71da-cdc3-4120-89e7-21ff59b441bf\"}],\"packageUris\":[\"http://schema.mathworks.com/mf0/Connector/R2020b\"],\"version\":\"1.0\"}"
  Vin+ : PMIOPort  Side=Left
  Vin- : PMIOPort  Port=2  Side=Left
  Vout+ : PMIOPort  Port=3  Side=Right
  Vout- : PMIOPort  Port=4  Side=Right
  meas : Outport

== system ConverterLibrary/Power Converter Plant/Soft-Switching Converters/LLC Converter/LLC Primary Inverter and Resonant Tank ==
  G : Inport
  LLC Detailed Model : Subsystem  VariantControl=DetailedModel
  LLC Simplified Model : Subsystem  VariantControl=SimplifiedModel
  + : PMIOPort  Side=Left
  - : PMIOPort  Port=2  Side=Left
  P2+ : PMIOPort  Port=3  Side=Right
  N2 : PMIOPort  Port=4  Side=Right
  P2- : PMIOPort  Port=5  Side=Right
  measInv : Outport
  measTank : Outport  Port=2

== system ConverterLibrary/Power Converter Plant/Soft-Switching Converters/LLC Converter/Rectifier ==
  C : fl_lib/Electrical/Electrical Elements/Capacitor  c=Cf F  r=Esr Ohm  g=1e-05 1/Ohm  i_specify=off  i_priority=None  i=0 A  i_nominal_specify=off  i_nominal_value=1  i_nominal_unit=A  v_specify=off  v_priority=None  v=450 V  v_nominal_specify=off  v_nominal_value=1  v_nominal_unit=V  vc_specify=on  vc_priority=High  vc=Vco_SI V  vc_nominal_specify=off  vc_nominal_value=1  vc_nominal_unit=V
  Iout : Subsystem
      mask Display: disp("I")
  IoutRect : Subsystem
      mask Display: disp("I")
  Rectifier Bridge : Subsystem  Variant=on  VariantControlMode=label  LabelModeActiveChoice=FullBridgeIdealDiode
  Subsystem4 : Subsystem
      settings: PortSchema="{\"entries\":[{\"content\":{\"sides\":[{\"content\":{\"connectorIds\":[\"LConn1\"]},\"type\":\"ConnectorPlacement.EquallySpacedRectSide\",\"uuid\":\"e749c2ff-fd60-426f-a769-b61a7dfe80d2\"},{\"content\":{\"connectorIds\":[\"RConn1\",\"Out1\"],\"side\":\"RIGHT\"},\"type\":\"ConnectorPlacement.EquallySpacedRectSide\",\"uuid\":\"f3bb02bd-f8d2-4326-b68c-6f969fa4ac22\"},{\"content\":{\"side\":\"TOP\"},\"type\":\"ConnectorPlacement.EquallySpacedRectSide\",\"uuid\":\"9ab7a0d1-20d8-49e4-8eb3-54d34434204c\"}]},\"type\":\"ConnectorPlacement.EquallySpacedConnector\",\"uuid\":\"19e2a6d5-13f4-47de-bb59-b826817cba83\"}],\"packageUris\":[\"http://schema.mathworks.com/mf0/Connector/R2020b\"],\"version\":\"1.0\"}"
      mask Display: disp("V")
  Vout : Subsystem
      settings: PortSchema="{\"entries\":[{\"content\":{\"sides\":[{\"content\":{\"connectorIds\":[\"LConn1\"]},\"type\":\"ConnectorPlacement.EquallySpacedRectSide\",\"uuid\":\"e749c2ff-fd60-426f-a769-b61a7dfe80d2\"},{\"content\":{\"connectorIds\":[\"RConn1\",\"Out1\"],\"side\":\"RIGHT\"},\"type\":\"ConnectorPlacement.EquallySpacedRectSide\",\"uuid\":\"f3bb02bd-f8d2-4326-b68c-6f969fa4ac22\"},{\"content\":{\"side\":\"TOP\"},\"type\":\"ConnectorPlacement.EquallySpacedRectSide\",\"uuid\":\"9ab7a0d1-20d8-49e4-8eb3-54d34434204c\"}]},\"type\":\"ConnectorPlacement.EquallySpacedConnector\",\"uuid\":\"19e2a6d5-13f4-47de-bb59-b826817cba83\"}],\"packageUris\":[\"http://schema.mathworks.com/mf0/Connector/R2020b\"],\"version\":\"1.0\"}"
      mask Display: disp("V")
  P+ : PMIOPort  Side=Left
  N : PMIOPort  Port=2  Side=Left
  P- : PMIOPort  Port=3  Side=Left
  + : PMIOPort  Port=4  Side=Right
  - : PMIOPort  Port=5  Side=Right
  Out Bus Element : Outport  PortName=meas  Element=Iout [A]
  BusElementOut : Outport  PortName=meas  Element=IL [A]
  BusElementOut1 : Outport  PortName=meas  Element=Vout [V]
  BusElementOut2 : Outport  PortName=meas  Element=Vac [V]
  BusElementOut3 : Outport  PortName=meas  Element=Is [A]
  wires:
  Iout/1(I) -> Out Bus Element/1
  IoutRect/1(I) -> BusElementOut/1
  Vout/1(V) -> BusElementOut1/1
  Subsystem4/1(V) -> BusElementOut2/1
  Rectifier Bridge/1(Ismeas) -> BusElementOut3/1
  connections:
  Rectifier Bridge/RConn1 -- IoutRect/LConn1
  N/RConn1 -- Rectifier Bridge/LConn2
  P-/RConn1 -- Rectifier Bridge/LConn3 -- Subsystem4/RConn1
  Rectifier Bridge/LConn1 -- Subsystem4/LConn1 -- P+/RConn1
  Vout/RConn1 -- C/RConn1 -- Rectifier Bridge/RConn2 -- -/RConn1
  Vout/LConn1 -- Iout/LConn1 -- IoutRect/RConn1 -- C/LConn1
  +/RConn1 -- Iout/RConn1

== system ConverterLibrary/Controller/Inverter-Based Resources/Grid-Forming Converter Controller/Current Limiting/CurrentLimitingMethod ==
  Igd : Inport
  Igq : Inport  Port=2
  currentLimitAndVirtual : Subsystem  VariantControl=both
  currentSaturation : Subsystem  VariantControl=ctSat
  virtualImpedance : Subsystem  VariantControl=virimp
  delVd : Outport
  delVq : Outport  Port=2
  Idmax : Outport  Port=3
  Iqmax : Outport  Port=4

== system ConverterLibrary/Controller/Inverter-Based Resources/Grid-Forming Converter Controller/Grid Voltage Reactive Power Support/Modifying Active Power Reference ==
  PrefInput : Inport
  Vd : Inport  Port=2
  Igd : Inport  Port=3
  Igq : Inport  Port=4
  AND : Logic  IconShape=distinctive  AllPortsSameDT=off  OutDataTypeStr=boolean
  Abs : Abs  SaturateOnIntegerOverflow=off
  Compare To Constant : simulink/Logic and Bit Operations/Compare To Constant  relop=<=  const=0.90  OutDataTypeStr=boolean
  Computing New Active Power Ref : Subsystem
  Math Function1 : Math  Operator=hypot
  Power Sign : Signum
  Product : Product
  Rate Transition1 : RateTransition
  Relay : Relay  OnSwitchValue=maxVICurrentLimit*0.96  OffSwitchValue=1
  Switch : Switch  Criteria=u2 > Threshold  SaturateOnIntegerOverflow=off  InputSameDT=off
  Pref : Outport
  wires:
  Rate Transition1/1 -> Relay/1
  Igq/1 -> Math Function1/1, Computing New Active Power Ref/1(Iq)
  Compare To Constant/1 -> AND/1
  AND/1 -> Switch/2
  Relay/1 -> AND/2
  Product/1 -> Pref/1
  Power Sign/1 -> Product/2
  Abs/1 -> Product/1
  Switch/1 -> Abs/1
  Igd/1 -> Math Function1/2
  PrefInput/1 -> Switch/3, Power Sign/1
  Vd/1 -> Compare To Constant/1, Computing New Active Power Ref/2(Vd)
  Math Function1/1 -> Rate Transition1/1  "Is"
  Computing New Active Power Ref/1(Pref) -> Switch/1

== system ConverterLibrary/Controller/Inverter-Based Resources/Grid-Forming Converter Controller/Grid Voltage Reactive Power Support/Modifying Reactive Power Reference ==
  Vgd : Inport
  Vgq : Inport  Port=2
  Qref : Inport  Port=3
  Pref : Inport  Port=4
  Changing the Power Reference : Subsystem
  Hysteresis : Subsystem
  Math Function : Math  Operator=hypot
  Merge : Merge
  Merge1 : Merge
  NOT : Logic  Operator=NOT  IconShape=distinctive  AllPortsSameDT=off  OutDataTypeStr=boolean
  Not Altering the Power Reference : Subsystem
  PrefNew : Outport
  QrefNew : Outport  Port=2
  wires:
  [Qref] -> Changing the Power Reference/4(Qref)
  [Pref] -> Changing the Power Reference/3(Pref)
  Merge/1 -> PrefNew/1
  Merge1/1 -> QrefNew/1
  Pref/1 -> [Pref], Not Altering the Power Reference/1(Pref)
  Vgq/1 -> Math Function/2
  Changing the Power Reference/2(Qrefv) -> Merge1/1
  [Vd] -> Changing the Power Reference/2(Vd)
  Hysteresis/1(LVFlag) -> NOT/1, Changing the Power Reference/Enable
  Qref/1 -> [Qref], Not Altering the Power Reference/2(Qref)
  NOT/1 -> Not Altering the Power Reference/Enable
  Changing the Power Reference/1(Prefv) -> Merge/1
  Not Altering the Power Reference/1(Prefv) -> Merge/2
  [Vs] -> Changing the Power Reference/1(Vs)
  Math Function/1 -> [Vs], Hysteresis/1(Vs)
  Not Altering the Power Reference/2(Qrefv) -> Merge1/2
  Vgd/1 -> Math Function/1, [Vd]

== system ConverterLibrary/Controller/Inverter-Based Resources/Grid-Forming Converter Controller/Measurement/Frequency Measurement ==
  Vabc : Inport
  Convert To PU : Gain  Gain=1/powerFreq
  Frequency Measurement : Subsystem  TreatAsAtomicUnit=on  SystemSampleTime=sampleTime  mask{initialFrequency=powerFreq, sampleTime=activePowerSampleTime}
      mask prompts: initialFrequency "Initial frequency in Hz"; sampleTime "Sample time in sec"
      mask DialogControl Container7 Prompt: General
  Low-Pass Filter : eeGeneralControl/Low-Pass Filter (Discrete or Continuous)  K=1  T=freqMeasTimeConst  B=inf  A=-inf  init_option=Inherited from block input  x0=0  Ts=-1
  Low-Pass Filter1 : eeGeneralControl/Low-Pass Filter (Discrete or Continuous)  K=1  T=0.1/powerFreq  B=inf  A=-inf  init_option=Inherited from block input  x0=0  Ts=-1
  Saturation : Saturate  UpperLimit=1.1  LowerLimit=0.9
  freq : Outport
  wires:
  Saturation/1 -> freq/1
  Low-Pass Filter1/1 -> Frequency Measurement/1(abc)
  Vabc/1 -> Low-Pass Filter1/1
  Convert To PU/1 -> Saturation/1
  Frequency Measurement/1(Freq) -> Low-Pass Filter/1
  Low-Pass Filter/1 -> Convert To PU/1  "Freq"

== system ConverterLibrary/Controller/Inverter-Based Resources/Grid-Forming Converter Controller/Measurement/abc2dq ==
  Igabc : Inport
  Angle : Inport  Port=2
  Vgabc : Inport  Port=3
  Supply Current to dq : Subsystem
  Supply Voltage  to dq : Subsystem
  Vgd : Outport
  Vgq : Outport  Port=2
  Igd : Outport  Port=3
  Igq : Outport  Port=4
  wires:
  Supply Voltage  to dq/2(Vgq) -> Vgq/1  "Vgq"
  Supply Voltage  to dq/1(Vgd) -> Vgd/1  "Vgd"
  Supply Current to dq/2(Igq) -> Igq/1  "Iq"
  Supply Current to dq/1(Igd) -> Igd/1  "Id"
  Igabc/1 -> Supply Current to dq/1(abc)
  Vgabc/1 -> Supply Voltage  to dq/2(abc)
  Angle/1 -> Supply Current to dq/2(Angle), Supply Voltage  to dq/1(Angle)

== system ConverterLibrary/Controller/Inverter-Based Resources/Grid-Forming Converter Controller/Power Control/ActivePowerControl ==
  Pref : Inport
  Pmeas : Inport  Port=2
  fgrid : Inport  Port=3
  droopControl : Subsystem  VariantControl=droop
  vsmControl : Subsystem  VariantControl=vsm
  Theta : Outport
  w : Outport  Port=2

== system ConverterLibrary/Controller/Inverter-Based Resources/Grid-Forming Converter Controller/Power Control/ReactiveControl ==
  note: Vs-delV
  Qref : Inport
  Qmeas : Inport  Port=2
  Constant : Constant  Value=voltreference
  Constant2 : Constant  Value=0
  Gain : Gain  Gain=QVoltDroop
  Low-Pass Filter (Discrete or Continuous) : eeGeneralControl/Low-Pass Filter (Discrete or Continuous)  K=1  T=QVoltFilterTC  B=inf  A=-inf  init_option=Specify as parameter  x0=0  Ts=activePowerSampleTime
  Product1 : Product
  Saturation1 : Saturate  UpperLimit=(dcBusVoltage/2)/(sqrt(2/3)*gridLineVoltage)  LowerLimit=-(dcBusVoltage/2)/(sqrt(2/3)*gridLineVoltage)
  Sum : Sum  Inputs=|+-
  Sum1 : Sum  Inputs=|++
  Vmd : Outport
  Vmq : Outport  Port=2
  wires:
  Saturation1/1 -> Vmd/1
  Qref/1 -> Sum/1
  Sum1/1 -> Product1/1
  Constant2/1 -> Vmq/1
  Constant/1 -> Sum1/2, Product1/2
  Product1/1 -> Saturation1/1  "Q"
  Gain/1 -> Sum1/1
  Low-Pass Filter (Discrete or Continuous)/1 -> Sum/2
  Qmeas/1 -> Low-Pass Filter (Discrete or Continuous)/1
  Sum/1 -> Gain/1
